simulink model "adaptive_kalman_like_1x1x1"  (R2023a)
settings: Solver=FixedStepAuto  StartTime=0.0  StopTime=40.0  RelTol=1e-3
values from neighbouring files (symbols this model uses):
  alpha = 0.9999    [Initialization_1x1x1.m]    (also in Initialization_1x2x2.m)
  B = 1    [Initialization_1x1x1.m]    (also in Initialization_1x2x2.m)
  F_n = 1.0001*eye(N)    [Initialization_1x1x1.m]
  fs = 1000    [Initialization_1x1x1.m]    (also in Initialization_1x2x2.m; Initialization_fxKalman.m; Initialization_path_estimation.m)
  K = 1    [Initialization_1x1x1.m]    (also in Initialization_1x2x2.m = 2; Initialization_fxKalman.m = 2)
  m = 4    [Initialization_fxKalman.m]
  N = L*I*J    (= 200)    [Initialization_1x1x1.m]    (also in Initialization_1x2x2.m; Initialization_fxKalman.m = 1)
  P = (5e-6)*eye(N)    [Initialization_1x1x1.m]    (also in Initialization_1x2x2.m; Initialization_fxKalman.m = (5e-6)*eye(M))
  Q = sigma_q^2*eye(N)    [Initialization_1x1x1.m]    (also in Initialization_1x2x2.m)
  Ts = 1/fs    (= 0.001)    [Initialization_1x1x1.m]    (also in Initialization_1x2x2.m; Initialization_fxKalman.m; Initialization_path_estimation.m)
undefined symbols (not defined in the file or in its folder): S1
libraries: speedgoatlib_IO104 x3, matrix_library x1, dspsrcs4 x1, simulink x1
settings Model: Creator=Tamida  LastModifiedBy=tislam
settings SolverCC: ConcurrentTasks=on  PositivePriorityOrder=on
settings OptimizationCC: BlockReduction=off  OptimizeBlockIOStorage=off
settings DebuggingCC: TasksWithSamePriorityMsg=none
settings HardwareCC: ProdBitPerLong=64  ProdLongLongMode=on  ProdHWDeviceType=Intel->x86-64 (Linux 64)
settings RTWCC: Description=Simulink Real-Time  SystemTargetFile=slrealtime.tlc  TemplateMakefile=slrealtime_default_tmf  Toolchain=Simulink Real-Time Toolchain  BuildConfiguration=Faster Runs  CodeExecutionProfiling=on  TargetLang=C++

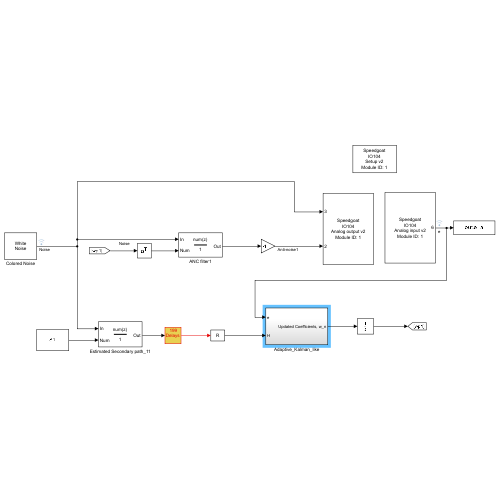
[thumbnail: Simulink's stored preview of the top-level diagram]
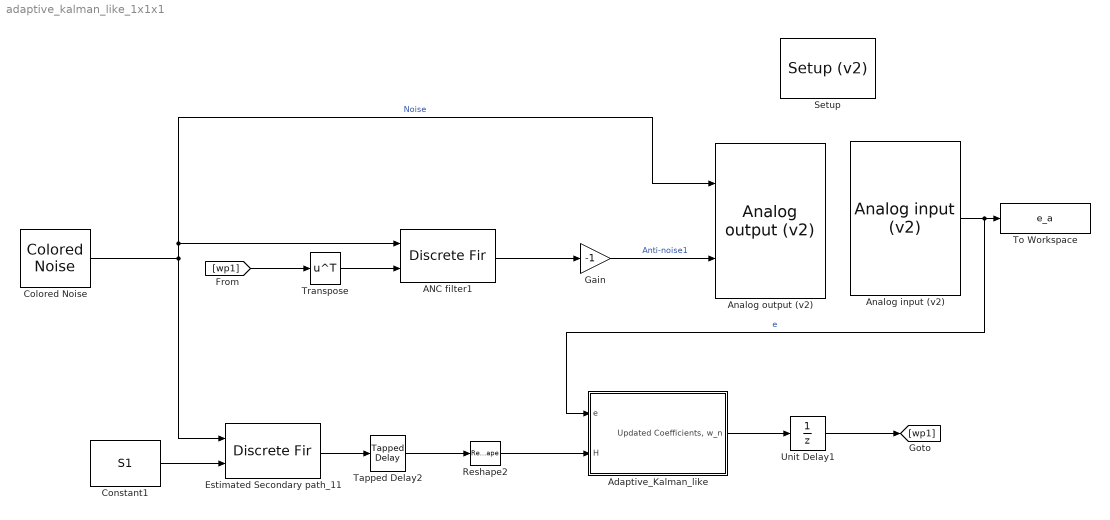
== system adaptive_kalman_like_1x1x1 ==
  ANC filter1 : DiscreteFir  CoefSource=Input port
      settings: InputPortMap=u0,u1
  Adaptive_Kalman_like : Subsystem
  "Analog input (v2) " : speedgoatlib_IO104/Analog input (v2)   parModuleId=1  parTs=1/fs  parPciSlot=-1  parAdChannels=6  parAdChannelsSorted=6  parAdRange1=+-2.5V  parAdRange2=+-2.5V  parAdCoupling=Differential  parAdFrameSize=1  parAdUseTrigger=off  parAdClockInitiator=Initiator  parAdSampleTime=1.000000000e-03  parTriggerInitiator=Initiator  parTriggerRate=-1.000000000e+00
      settings: SourceProductName=Simulink Real-Time: Speedgoat I/O Blockset
  "Analog output (v2) " : speedgoatlib_IO104/Analog output (v2)   parModuleId=1  parTs=1/fs  parPciSlot=-1  parDaSimultaneous=on  parDaChannels=[3,2]  parDaChannelsSorted=[2,3]  parDaInitValue=[0,0]  parDaReset=[1,1]  parDaRange=+-2.5V  parDaFrameSize=1  parDaUseTrigger=off  parDaClockInitiator=Initiator  parDaSampleTime=1.000000000e-03  parTriggerInitiator=Initiator  parTriggerRate=-1.000000000e+00  parAdBlockPresent=1
      settings: SourceProductName=Simulink Real-Time: Speedgoat I/O Blockset
  Colored Noise : dspsrcs4/Colored Noise  Color=white  InverseFrequencyPower=1  BoundedOutput=on  NumChannels=1  OutputDataType=double  SamplesPerFrame=1  SampleTime=Ts  RandomStream=mt19937ar with seed  Seed=67  SimulateUsing=Interpreted execution
      settings: LibrarySourceBlock=audiosources/Colored Noise
  Constant1 : Constant  Value=S1  SampleTime=-1
  Estimated Secondary path_11 : DiscreteFir  CoefSource=Input port  Coefficients=[-1.6 -0.6 -.25 0.4 -1.5 0.4 -1.2 0.07 0.6 0.3]
      settings: InputPortMap=u0,u1
  Gain : Gain  Gain=-1
  Reshape2 : Reshape  OutputDimensionality=Customize  OutputDimensions=[K*B,N]
  Setup : speedgoatlib_IO104/Setup (v2)   parPciSlot=-1  parModuleId=1  parTriggerInitiator=Initiator  parTriggerRate=1/fs  parCalibrate=on  parAdChannels=[6]  parAdRange1=+-2.5V  parAdRange2=+-2.5V  parAdCoupling=Differential  parAdUseTrigger=off  parAdFrameSize=1  parAdClockInitiator=Initiator  parAdSampleTime=1/fs  parDaSimultaneous=on  parDaChannels=[3 2]  parDaChannelsSorted=[2,3]  parDaInitValue=[0]  parDaReset=[1]  parDaRange=+-2.5V  parDaUseTrigger=off  parDaFrameSize=1  parDaClockInitiator=Initiator  parDaSampleTime=1/fs  parDioByte0Dir=Outputs  parDioByte1Dir=Inputs  parDoChannels=0  parDoInitValues=[0]  parDoReset=[1]  parDiChannels=0
      settings: SourceProductName=Simulink Real-Time: Speedgoat I/O Blockset
  Tapped Delay2 : simulink/Discrete/Tapped Delay  vinit=0.0  samptime=-1  NumDelays=(K*B*N)-1  DelayOrder=Newest  includeCurrent=on
  To Workspace : ToWorkspace  VariableName=e_a  SaveFormat=Structure With Time  SampleTime=-1
  Transpose : Math  Operator=transpose
  Unit Delay1 : UnitDelay  SampleTime=Ts  HasFrameUpgradeWarning=on
  wires:
  Tapped Delay2/1 -> Reshape2/1
  Estimated Secondary path_11/1 -> Tapped Delay2/1
  Constant1/1 -> Estimated Secondary path_11/2
  Reshape2/1 -> Adaptive_Kalman_like/2(H)
  [wp1] -> Transpose/1
  Transpose/1 -> ANC filter1/2
  ANC filter1/1 -> Gain/1
  Colored Noise/1 -> "Analog output (v2) "/1, ANC filter1/1, Estimated Secondary path_11/1  "Noise"
  Adaptive_Kalman_like/1("Updated Coefficients, w_n") -> Unit Delay1/1
  Unit Delay1/1 -> [wp1]
  Gain/1 -> "Analog output (v2) "/2  "Anti-noise1"
  "Analog input (v2) "/1 -> To Workspace/1, Adaptive_Kalman_like/1(e)  "e"

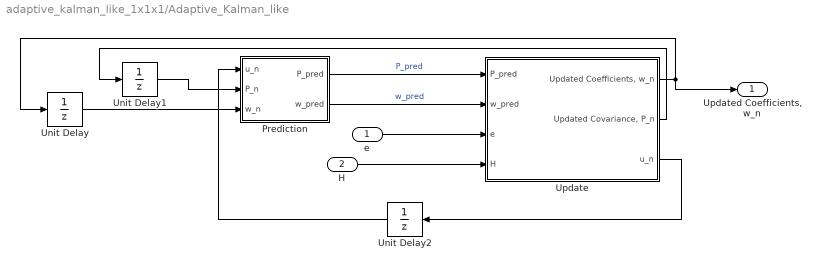
== system adaptive_kalman_like_1x1x1/Adaptive_Kalman_like ==
  e : Inport
  H : Inport  Port=2
  Prediction : Subsystem
  Unit Delay : UnitDelay  InitialCondition=m  SampleTime=Ts  HasFrameUpgradeWarning=on
  Unit Delay1 : UnitDelay  InitialCondition=P  SampleTime=Ts  HasFrameUpgradeWarning=on
  Unit Delay2 : UnitDelay  SampleTime=-1  HasFrameUpgradeWarning=on
  Update : Subsystem
  "Updated Coefficients, w_n" : Outport
  wires:
  Prediction/1(P_pred) -> Update/1(P_pred)  "P_pred"
  H/1 -> Update/4(H)
  e/1 -> Update/3(e)
  Prediction/2(w_pred) -> Update/2(w_pred)  "w_pred"
  Update/2("Updated Covariance, P_n") -> Unit Delay1/1
  Update/1("Updated Coefficients, w_n") -> "Updated Coefficients, w_n"/1, Unit Delay/1
  Update/3(u_n) -> Unit Delay2/1
  Unit Delay2/1 -> Prediction/1(u_n)
  Unit Delay/1 -> Prediction/3(w_n)
  Unit Delay1/1 -> Prediction/2(P_n)

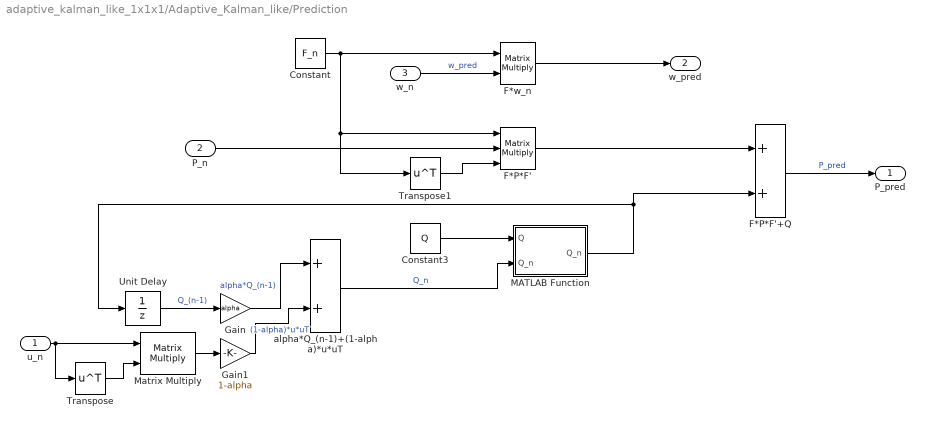
== system adaptive_kalman_like_1x1x1/Adaptive_Kalman_like/Prediction ==
  u_n : Inport
  P_n : Inport  Port=2
  w_n : Inport  Port=3
  Constant : Constant  Value=F_n
  Constant3 : Constant  Value=Q
  F*P*F' : Product  Inputs=3  Multiplication=Matrix(*)
  F*P*F'+Q : Sum  InputSameDT=on  OutDataTypeStr=Inherit: Inherit via back propagation
  F*w_n : Product  Multiplication=Matrix(*)
  Gain : Gain  Gain=alpha
  Gain1 : Gain  Gain=1-alpha
  MATLAB Function : MATLAB Function  TreatAsAtomicUnit=on
  Matrix Multiply : Product  Multiplication=Matrix(*)
  Transpose : Math  Operator=transpose
  Transpose1 : Math  Operator=transpose
  Unit Delay : UnitDelay  SampleTime=-1  HasFrameUpgradeWarning=on
  alpha*Q_(n-1)+(1-alpha)*u*uT : Sum  InputSameDT=on  OutDataTypeStr=Inherit: Inherit via back propagation
  P_pred : Outport
  w_pred : Outport  Port=2
  wires:
  MATLAB Function/1(Q_n) -> F*P*F'+Q/2, Unit Delay/1
  Constant3/1 -> MATLAB Function/1(Q)
  Unit Delay/1 -> Gain/1  "Q_(n-1)"
  Gain/1 -> alpha*Q_(n-1)+(1-alpha)*u*uT/1  "alpha*Q_(n-1)"
  Gain1/1 -> alpha*Q_(n-1)+(1-alpha)*u*uT/2  "(1-alpha)*u*uT"
  alpha*Q_(n-1)+(1-alpha)*u*uT/1 -> MATLAB Function/2("Q_n ")  "Q_n"
  Matrix Multiply/1 -> Gain1/1
  u_n/1 -> Transpose/1, Matrix Multiply/1
  Transpose/1 -> Matrix Multiply/2
  P_n/1 -> F*P*F'/2
  F*w_n/1 -> w_pred/1
  F*P*F'+Q/1 -> P_pred/1  "P_pred"
  w_n/1 -> F*w_n/2  "w_pred"
  F*P*F'/1 -> F*P*F'+Q/1
  Transpose1/1 -> F*P*F'/3
  Constant/1 -> Transpose1/1, F*P*F'/1, F*w_n/1

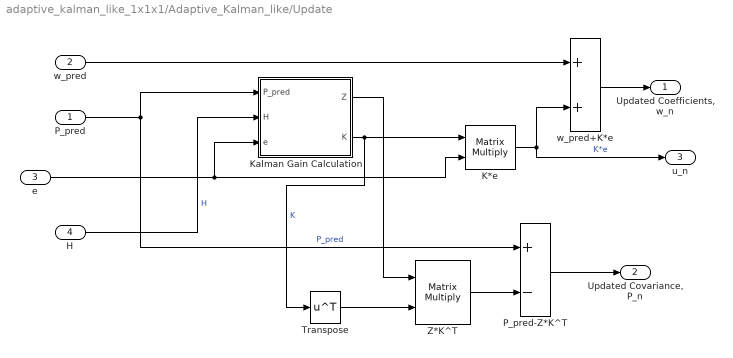
== system adaptive_kalman_like_1x1x1/Adaptive_Kalman_like/Update ==
  P_pred : Inport
  w_pred : Inport  Port=2
  e : Inport  Port=3
  H : Inport  Port=4
  K*e : Product  Multiplication=Matrix(*)  InputSameDT=on  OutDataTypeStr=Inherit: Inherit via back propagation
  Kalman Gain Calculation : Subsystem
  P_pred-Z*K^T : Sum  Inputs=+-  InputSameDT=on  OutDataTypeStr=Inherit: Inherit via back propagation
  Transpose : Math  Operator=transpose
  Z*K^T : Product  Multiplication=Matrix(*)  InputSameDT=on  OutDataTypeStr=Inherit: Same as first input
  w_pred+K*e : Sum  InputSameDT=on  OutDataTypeStr=Inherit: Inherit via back propagation
  "Updated Coefficients, w_n" : Outport
  "Updated Covariance, P_n" : Outport  Port=2
  u_n : Outport  Port=3
  wires:
  P_pred/1 -> Kalman Gain Calculation/1(P_pred), P_pred-Z*K^T/1  "P_pred"
  Kalman Gain Calculation/2(K) -> K*e/1, Transpose/1  "K"
  Z*K^T/1 -> P_pred-Z*K^T/2
  K*e/1 -> w_pred+K*e/2, u_n/1  "K*e"
  e/1 -> Kalman Gain Calculation/3(e), K*e/2
  w_pred+K*e/1 -> "Updated Coefficients, w_n"/1
  H/1 -> Kalman Gain Calculation/2(H)  "H"
  w_pred/1 -> w_pred+K*e/1
  P_pred-Z*K^T/1 -> "Updated Covariance, P_n"/1
  Kalman Gain Calculation/1(Z) -> Z*K^T/1
  Transpose/1 -> Z*K^T/2

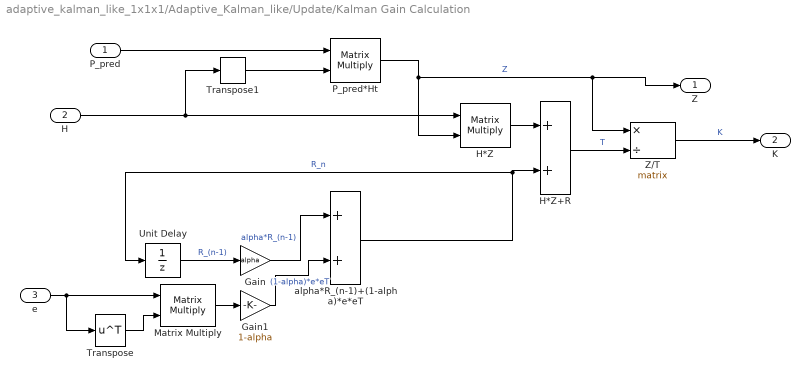
== system adaptive_kalman_like_1x1x1/Adaptive_Kalman_like/Update/Kalman Gain Calculation ==
  P_pred : Inport
  H : Inport  Port=2
  e : Inport  Port=3
  Gain : Gain  Gain=alpha
  Gain1 : Gain  Gain=1-alpha
  H*Z : Product  Multiplication=Matrix(*)  InputSameDT=on  OutDataTypeStr=Inherit: Inherit via back propagation
  H*Z+R : Sum  InputSameDT=on  OutDataTypeStr=Inherit: Inherit via back propagation
  Matrix Multiply : Product  Multiplication=Matrix(*)
  P_pred*Ht : Product  Multiplication=Matrix(*)  InputSameDT=on  OutDataTypeStr=Inherit: Inherit via back propagation
  Transpose : Math  Operator=transpose
  Transpose1 : matrix_library/Transpose
  Unit Delay : UnitDelay  SampleTime=-1  HasFrameUpgradeWarning=on
  Z/T : Product  Inputs=*/  Multiplication=Matrix(*)
  alpha*R_(n-1)+(1-alpha)*e*eT : Sum  InputSameDT=on  OutDataTypeStr=Inherit: Inherit via back propagation
  Z : Outport
  K : Outport  Port=2
  wires:
  H/1 -> H*Z/1, Transpose1/1
  H*Z/1 -> H*Z+R/1
  H*Z+R/1 -> Z/T/2  "T"
  P_pred/1 -> P_pred*Ht/1
  P_pred*Ht/1 -> Z/1, Z/T/1, H*Z/2  "Z"
  Transpose1/1 -> P_pred*Ht/2
  Z/T/1 -> K/1  "K"
  Matrix Multiply/1 -> Gain1/1
  e/1 -> Matrix Multiply/1, Transpose/1
  Transpose/1 -> Matrix Multiply/2
  Gain1/1 -> alpha*R_(n-1)+(1-alpha)*e*eT/2  "(1-alpha)*e*eT"
  Unit Delay/1 -> Gain/1  "R_(n-1)"
  alpha*R_(n-1)+(1-alpha)*e*eT/1 -> Unit Delay/1, H*Z+R/2  "R_n"
  Gain/1 -> alpha*R_(n-1)+(1-alpha)*e*eT/1  "alpha*R_(n-1)"

== matlab function adaptive_kalman_like_1x1x1/Adaptive_Kalman_like/Prediction/MATLAB Function ==
  data: Q input; Q_n output; Q_n input
function Q_n  = fcn(Q, Q_n)

%#codegen
if Q_n<Q
    Q_n = Q; 
else
    Q_n = Q_n;
end
